simulink model "LQG"  (R2025b)
settings: Solver=VariableStepAuto  StartTime=0.0  StopTime=10.0  RelTol=1e-3
undefined symbols (not defined in the file): b, C, c, g, I, kb, KK, kt, l, M, m, r, Rm, sysKF
libraries: simulink x5
settings Model: Creator=Usuario  LastModifiedBy=joelalfaro

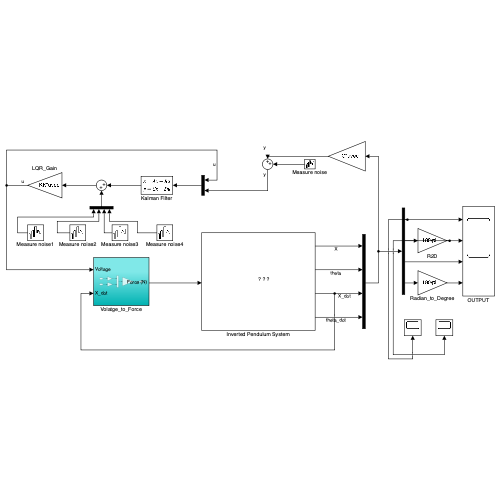
[thumbnail: Simulink's stored preview of the top-level diagram]
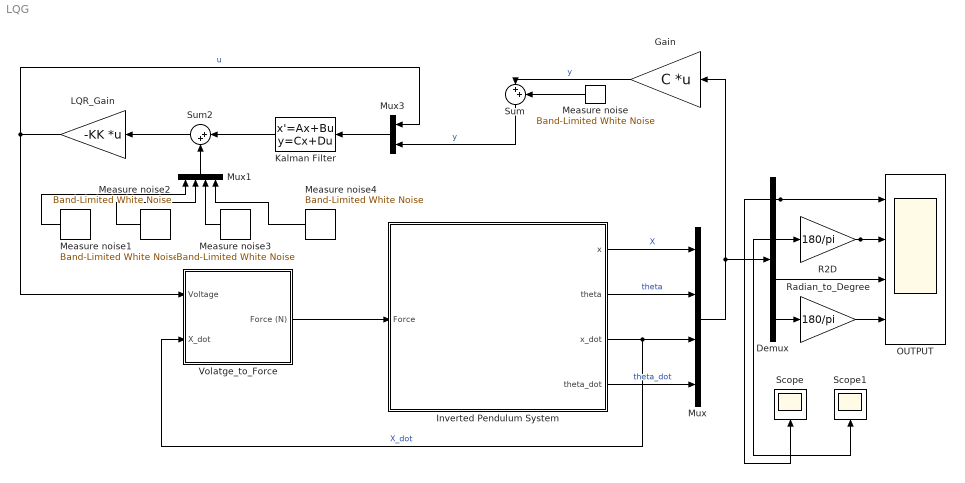
== system LQG ==
  Demux : Demux
  Gain : Gain  Gain=C  Multiplication=Matrix(K*u) (u vector)
  Inverted Pendulum System : Subsystem
      mask Display: image('ip_model.png');
  Kalman Filter : StateSpace  A=sysKF.A  B=sysKF.B  C=sysKF.C  D=sysKF.D  InitialCondition=0
  LQR_Gain : Gain  Gain=-KK  Multiplication=Matrix(K*u) (u vector)
  Measure noise{,1..4} (5 alike) : simulink/Sources/Band-Limited White Noise  Cov=[0.05]  Ts=1  seed=[23341]
  Mux : Mux
  Mux1 : Mux
  Mux3 : Mux  Inputs=2
  OUTPUT : Scope  NumInputPorts=4
      settings: ActiveDisplayString=4  ActiveDisplayYMinimum=-175.01239944867373  ActiveDisplayYMaximum=256.9962748777549  YLabel=\theta dot (deg/sec)  DataLoggingVariableName=ScopeData2
  R2D : Gain  Gain=180/pi
  Radian_to_Degree : Gain  Gain=180/pi
  Scope : Scope
      settings: ActiveDisplayYMinimum=0.030577971114128383  ActiveDisplayYMaximum=0.77691598435844667
  Scope1 : Scope
      settings: ActiveDisplayYMinimum=151.06879516577567  ActiveDisplayYMaximum=200.28914353055384
  Sum : Sum  Inputs=|++
  Sum2 : Sum  Inputs=|++
  Volatge_to_Force : Subsystem
  wires:
  Inverted Pendulum System/2(theta) -> Mux/2  "theta"
  Demux/2 -> R2D/1
  Demux/3 -> OUTPUT/3
  Demux/1 -> OUTPUT/1, Scope/1
  Mux/1 -> Demux/1, Gain/1
  Inverted Pendulum System/3(x_dot) -> Volatge_to_Force/2(X_dot), Mux/3  "X_dot"
  R2D/1 -> OUTPUT/2, Scope1/1
  Radian_to_Degree/1 -> OUTPUT/4
  Volatge_to_Force/1(Force (N)) -> Inverted Pendulum System/1(Force)
  Inverted Pendulum System/4(theta_dot) -> Mux/4  "theta_dot"
  Inverted Pendulum System/1(x) -> Mux/1  "X"
  Demux/4 -> Radian_to_Degree/1
  Measure noise/1 -> Sum/2
  LQR_Gain/1 -> Mux3/1, Volatge_to_Force/1(Voltage)  "u"
  Mux3/1 -> Kalman Filter/1
  Gain/1 -> Sum/1  "y"
  Sum/1 -> Mux3/2  "y"
  Measure noise1/1 -> Mux1/1
  Measure noise2/1 -> Mux1/2
  Measure noise4/1 -> Mux1/4
  Measure noise3/1 -> Mux1/3
  Sum2/1 -> LQR_Gain/1
  Kalman Filter/1 -> Sum2/1
  Mux1/1 -> Sum2/2

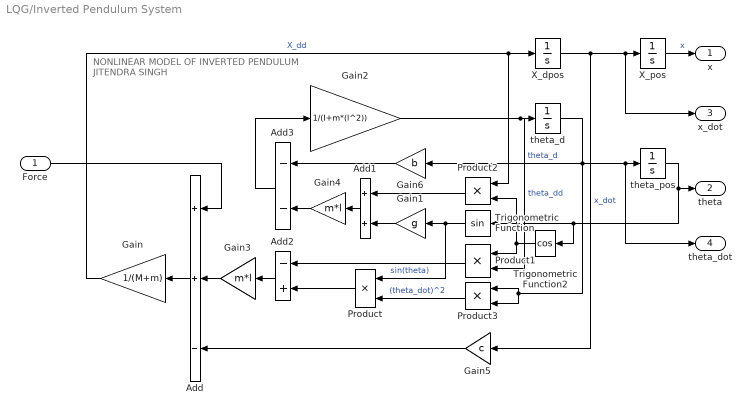
== system LQG/Inverted Pendulum System ==
  note: NONLINEAR MODEL OF
      | INVERTED PENDULUM
      | JITENDRA SINGH
  Force : Inport
  Add : Sum  Inputs=++-
  Add1 : Sum
  Add2 : Sum  Inputs=-+
  Add3 : Sum  Inputs=--
  Gain : Gain  Gain=1/(M+m)
  Gain1 : Gain  Gain=g
  Gain2 : Gain  Gain=1/(I+m*(l^2))
  Gain3 : Gain  Gain=m*l
  Gain4 : Gain  Gain=m*l
  Gain5 : Gain  Gain=c
  Gain6 : Gain  Gain=b
  Product{,1..3} (4 alike) : Product
  Trigonometric Function : Trigonometry
  Trigonometric Function2 : Trigonometry  Operator=cos
  X_dpos : Integrator
  X_pos : Integrator  InitialCondition=0.2
  theta_d : Integrator
  theta_pos : Integrator  InitialCondition=160*(pi/180)
  x : Outport  VectorParamsAs1DForOutWhenUnconnected=off
  theta : Outport  Port=2  VectorParamsAs1DForOutWhenUnconnected=off
  x_dot : Outport  Port=3  VectorParamsAs1DForOutWhenUnconnected=off
  theta_dot : Outport  Port=4  VectorParamsAs1DForOutWhenUnconnected=off
  wires:
  Gain5/1 -> Add/3
  Add2/1 -> Gain3/1
  Add3/1 -> Gain2/1
  Trigonometric Function2/1 -> Product2/2, Product1/1
  Trigonometric Function/1 -> Product/1, Gain1/1  "sin(theta)"
  Gain3/1 -> Add/2
  theta_d/1 -> Product3/2, Product3/1, Gain6/1, theta_dot/1, theta_pos/1  "theta_d"
  Product2/1 -> Add1/1
  Product/1 -> Add2/2
  Gain4/1 -> Add3/2
  Product3/1 -> Product/2  "(theta_dot)^2"
  X_pos/1 -> x/1  "x"
  Product1/1 -> Add2/1
  Gain/1 -> X_dpos/1, Product2/1  "X_dd"
  Add/1 -> Gain/1
  Gain2/1 -> Product1/2, theta_d/1  "theta_dd"
  Gain6/1 -> Add3/1
  theta_pos/1 -> Trigonometric Function2/1, Trigonometric Function/1, theta/1
  Force/1 -> Add/1
  Gain1/1 -> Add1/2
  X_dpos/1 -> x_dot/1, X_pos/1, Gain5/1  "x_dot"
  Add1/1 -> Gain4/1

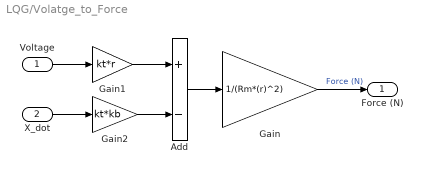
== system LQG/Volatge_to_Force ==
  Voltage : Inport
  X_dot : Inport  Port=2
  Add : Sum  Inputs=+-
  Gain : Gain  Gain=1/(Rm*(r)^2)
  Gain1 : Gain  Gain=kt*r
  Gain2 : Gain  Gain=kt*kb
  Force (N) : Outport  VectorParamsAs1DForOutWhenUnconnected=off
  wires:
  Gain1/1 -> Add/1
  Gain2/1 -> Add/2
  Voltage/1 -> Gain1/1
  Gain/1 -> Force (N)/1  "Force (N)"
  X_dot/1 -> Gain2/1
  Add/1 -> Gain/1
